simulink model "PMSM_Simulation_2025a"  (R2025a)
settings: Solver=FixedStepDiscrete  StartTime=0.0  StopTime=10.0  FixedStep=0.00005/200  RelTol=1e-3
values from neighbouring files (symbols this model uses):
  MC_DCurrLopKi_CFG = 0.008293758    [PMSM_MC_Data_2025a.sldd]
  MC_DCurrLopKp_CFG = 0.0870848    [PMSM_MC_Data_2025a.sldd]
  MC_MotModeDebug_CFG = 255.0    [PMSM_MC_Data_2025a.sldd]
  MC_POLE_NUM_CFG = 7.0    [PMSM_MC_Data_2025a.sldd]
  MC_QCurrLopKi_CFG = 0.008293758    [PMSM_MC_Data_2025a.sldd]
  MC_QCurrLopKp_CFG = 0.0870848    [PMSM_MC_Data_2025a.sldd]
  MC_SpdLopKi_CFG = 1.0E-5    [PMSM_MC_Data_2025a.sldd]
  MC_SpdLopKp_CFG = 0.002    [PMSM_MC_Data_2025a.sldd]
libraries: simulink x13, slpidlib x3, spsDCVoltageSourceLib x1, spsPermanentMagnetSynchronousMachineLib x1, spsUniversalBridgeLib x1, sps_lib x1
(part 2 of 2)

== system PMSM_Simulation_2025a/PMSM_MC/MC_HighFrqTask/FOC/SVPWM/SevenSegSVPWM/XYZCaculate ==
  Ualpha : Inport
  Ubeta : Inport  Port=2
  Udc : Inport  Port=3
  Ts : Inport  Port=4
  Add : Sum
  Add1 : Sum  Inputs=+-
  Fcn : Fcn  Expr=1/u
  Gain : Gain  Gain=3/2
  Gain1 : Gain  Gain=sqrt(3)
  Gain2 : Gain  Gain=sqrt(3)/2
  Mux : Mux  Inputs=3
  Product{,1..3} (4 alike) : Product
  XYZ : Outport
  wires:
  Ualpha/1 -> Gain/1
  Ubeta/1 -> Gain2/1, Gain1/1
  Gain/1 -> Add/2, Add1/2
  Gain1/1 -> Product/1
  Gain2/1 -> Add1/1, Add/1
  Ts/1 -> Product3/1
  Product3/1 -> Product1/2, Product/2, Product2/2
  Add/1 -> Product1/1
  Udc/1 -> Fcn/1
  Fcn/1 -> Product3/2
  Add1/1 -> Product2/1
  Product1/1 -> Mux/2
  Product2/1 -> Mux/3
  Product/1 -> Mux/1
  Mux/1 -> XYZ/1

== stateflow chart PMSM_Simulation_2025a/PMSM_MC/MC_LowFrqTask/MotModeCtr/Chart ==
  state Calibrate
    state Init
      en:
      MotCtrMode=0;
    state Calibrate1
      en:
      MotCtrMode=1;
      MotCalThetae = 0;//0°
    state Calibrate2
      en:
      MotOffsetBuff[0]=Ecode_cnt;
      MotCtrMode=2;
      MotCalThetae = 0;//0°
    state RngChk
      en:
      MotOffsetBuff[1]=Ecode_cnt;
      RangeCheck();
    (default) -> Init
    Init -> Calibrate1 : [MotorSpdRef != 0]
    Calibrate1 -> Calibrate2 : [after(1.5,sec)]
    Calibrate2 -> RngChk : [after(1.5,sec)]
  state RangeCheck [function]
    (default) -> (junction 21)
    (junction 21) -> (junction 23) [order 1] : [abs(MotOffsetBuff[0]-MotOffsetBuff[1])>100]
    (junction 21) -> (junction 24) [order 2] : {
        | MotCalNormal=1;
        | MotOffset = (MotOffsetBuff[0]+MotOffsetBuff[1])/2;
        | }
    (junction 23) -> (junction 25) : {MotCalNormal=0;}
    (junction 25) -> (junction 24)
    (junction 24) -> (junction 35)
  state CalFailed
    en:
    MotCtrMode=3;
  state Normal
    state Stop
      en:
      MotCtrMode=4;
    state Run
      en:
      MotCtrMode=5;
    (default) -> Stop
    Run -> Stop : [MotorSpdRef==0]
    Stop -> Run : [MotorSpdRef!=0]
  (default) -> Calibrate
  CalFailed -> Calibrate : [MotorSpdRef==0]
  RngChk -> CalFailed [order 1] : [MotCalNormal==0]
  RngChk -> Normal [order 2] : [MotCalNormal==1]
  data: MotCtrMode output uint8; Ecode_cnt input int32; MotorSpdRef input int16; MotOffset output int32; MotCalThetae output single; MotOffsetBuff local int32 size=2; MotCalNormal local boolean

== stateflow chart PMSM_Simulation_2025a/Scheduler ==
  (default) -> (junction 6)
  (junction 6) -> (junction 11) [order 1] : [counter%%4000==3999]
  (junction 6) -> (junction 10) [order 2]
  (junction 11) -> (junction 9) : {trig_MidFrq_1ms;}
  (junction 9) -> (junction 10)
  (junction 10) -> (junction 36)
  (junction 36) -> (junction 38) [order 1] : [counter%%200==199]
  (junction 36) -> (junction 41) [order 2]
  (junction 38) -> (junction 40) : {trig_HighFrq_50us;}
  (junction 40) -> (junction 41)
  (junction 41) -> (junction 18)
  (junction 18) -> (junction 20) [order 1] : [counter>=100000000]
  (junction 18) -> (junction 24) [order 2] : {counter++;}
  (junction 20) -> (junction 22) : {counter=0;}
  (junction 22) -> (junction 24)
  (junction 24) -> (junction 27)
  data: counter local uint32 =0
  events: trig_MidFrq_1ms output FUNCTION_CALL_EVENT; trig_HighFrq_50us output FUNCTION_CALL_EVENT
